simulink model "chaine_cbs"  (R2023b)
settings: Solver=FixedStepDiscrete  StartTime=0.0  StopTime=100000  FixedStep=1  RelTol=1e-3
values from neighbouring files (symbols this model uses):
  graine = round(P.graine)    [Parametres.m]    (also in Partie2.m = P.graine; parametres_perso.m = mod(sum(c .* (1:numel(c)) * 31) + 7 * numel(c), 2^31 - 1))
  p1 = P.p1    [Parametres.m]    (also in Partie2.m)
  pe = P.pe_cbs    [Parametres.m]
settings Model: Creator=e2403517  LastModifiedBy=e2403517

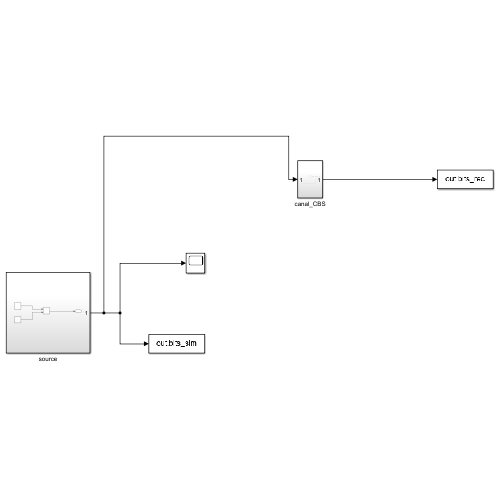
[thumbnail: Simulink's stored preview of the top-level diagram]
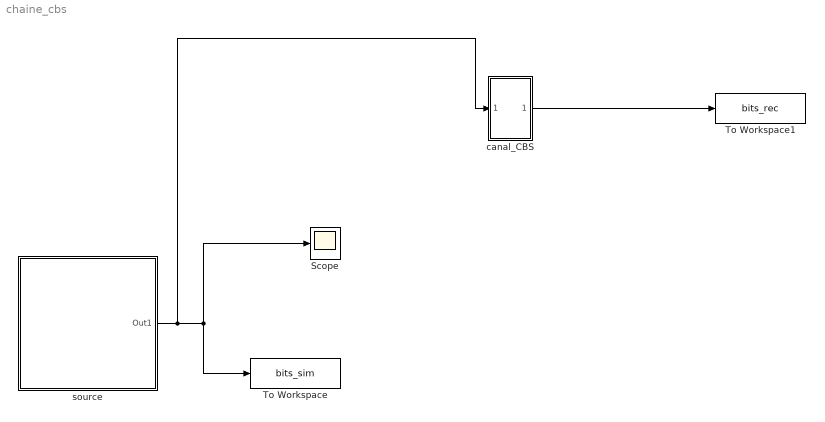
== system chaine_cbs ==
  Scope : Scope
  To Workspace : ToWorkspace  VariableName=bits_sim  SampleTime=1
  To Workspace1 : ToWorkspace  VariableName=bits_rec  SampleTime=1
  canal_CBS : Subsystem
  source : Subsystem
  wires:
  source/1(Out1) -> canal_CBS/1(In1), Scope/1, To Workspace/1
  canal_CBS/1(Out1) -> To Workspace1/1

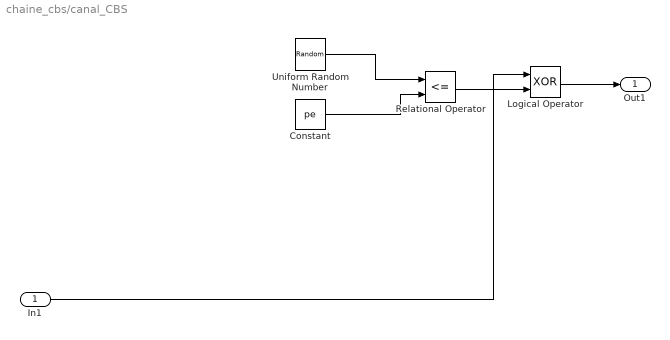
== system chaine_cbs/canal_CBS ==
  In1 : Inport
  Constant : Constant  Value=pe  SampleTime=1
  Logical Operator : Logic  Operator=XOR  AllPortsSameDT=off  OutDataTypeStr=boolean
  Relational Operator : RelationalOperator  Operator=<=  OutDataTypeStr=boolean  RndMeth=Simplest  InputSameDT=off
  Uniform Random Number : UniformRandomNumber  Minimum=0  Seed=graine+1  SampleTime=1
  Out1 : Outport
  wires:
  Relational Operator/1 -> Logical Operator/2
  Logical Operator/1 -> Out1/1
  Constant/1 -> Relational Operator/2
  Uniform Random Number/1 -> Relational Operator/1
  In1/1 -> Logical Operator/1

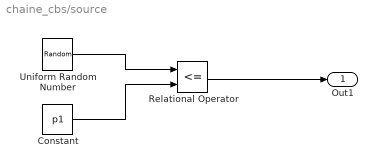
== system chaine_cbs/source ==
  Constant : Constant  Value=p1  SampleTime=1
  Relational Operator : RelationalOperator  Operator=<=  OutDataTypeStr=boolean  RndMeth=Simplest  InputSameDT=off
  Uniform Random Number : UniformRandomNumber  Minimum=0  Seed=graine  SampleTime=1
  Out1 : Outport
  wires:
  Uniform Random Number/1 -> Relational Operator/1
  Constant/1 -> Relational Operator/2
  Relational Operator/1 -> Out1/1
